simulink model "Main"  (R2025a)
settings: Solver=VariableStepAuto  StartTime=0.0  StopTime=inf  RelTol=1e-3
libraries: dspstat3 x21, simulink_extras x2, fuzblock x1
settings Model: Creator=felix  LastModifiedBy=felix

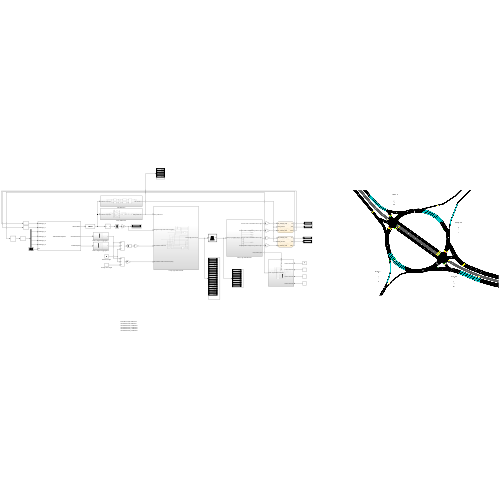
[thumbnail: Simulink's stored preview of the top-level diagram]
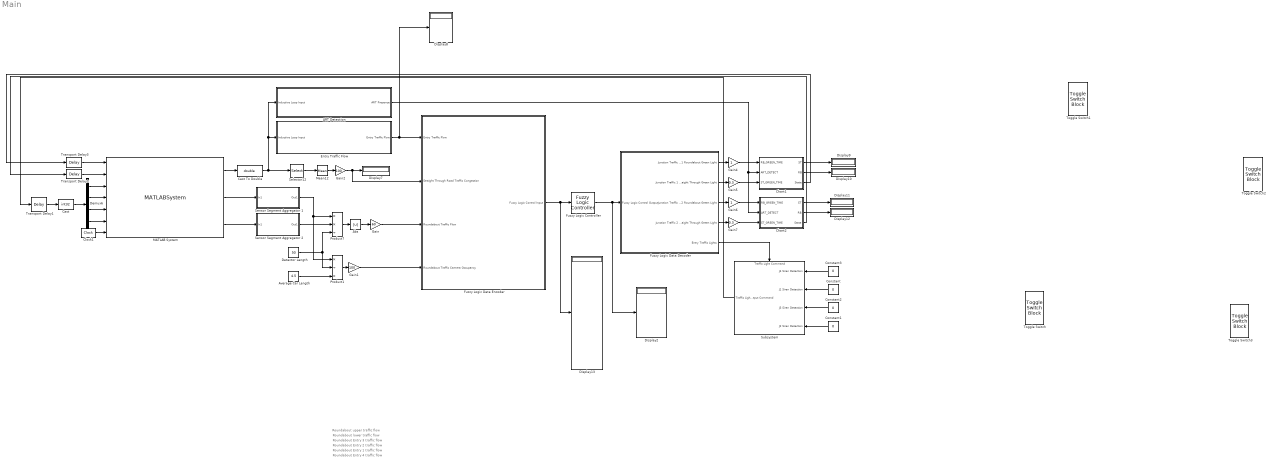
== system Main ==
  note: Roundabout Entry 4 traffic flow
  note: Roundabout Entry 1 traffic flow
  note: Roundabout Entry 2 traffic flow
  note: Roundabout Entry 3 traffic flow
  note: Roundabout lower traffic flow
  note: Roundabout upper traffic flow
  ART Detection : Subsystem
  Abs : Abs  SaturateOnIntegerOverflow=off
  Average Car Length : Constant  Value=4.5
  Cast : DataTypeConversion  OutDataTypeStr=int32  SaturateOnIntegerOverflow=off  RndMeth=Floor
  Cast To Double : DataTypeConversion  OutDataTypeStr=double  SaturateOnIntegerOverflow=off  RndMeth=Floor
  Chart1 : Stateflow chart  TreatAsAtomicUnit=on
      settings: PortSchema="{\"entries\":[{\"content\":{\"sides\":[{\"content\":{\"connectorIds\":[\"In1\",\"In3\",\"In2\"]},\"type\":\"ConnectorPlacement.EquallySpacedRectSide\",\"uuid\":\"637e66cb-ca59-4601-bc87-d398030e3d4e\"},{\"content\":{\"connectorIds\":[\"Out1\",\"Out2\",\"Out3\"],\"side\":\"RIGHT\"},\"type\":\"ConnectorPlacement.EquallySpacedRectSide\",\"uuid\":\"e38eed65-4b8e-4656-a325-0944c1a393f4\"},{\"content\":{\"side\":\"TOP\"},\"type\":\"ConnectorPlacement.EquallySpacedRectSide\",\"uuid\":\"0e3a8e04-edc4-4c67-baf8-ce5088455846\"}]},\"type\":\"ConnectorPlacement.EquallySpacedConnector\",\"uuid\":\"3222c7f8-a245-402d-95e3-93e9ec8df21d\"}],\"packageUris\":[\"http://schema.mathworks.com/mf0/Connector/R2020b\"],\"version\":\"1.0\"}"
  Chart2 : Stateflow chart  TreatAsAtomicUnit=on
      settings: PortSchema="{\"entries\":[{\"content\":{\"sides\":[{\"content\":{\"connectorIds\":[\"In1\",\"In3\",\"In2\"]},\"type\":\"ConnectorPlacement.EquallySpacedRectSide\",\"uuid\":\"3ce13be8-2b6b-44a6-8be1-1e74bcb078bf\"},{\"content\":{\"connectorIds\":[\"Out1\",\"Out2\",\"Out3\"],\"side\":\"RIGHT\"},\"type\":\"ConnectorPlacement.EquallySpacedRectSide\",\"uuid\":\"50de3ca6-7955-42e3-b87c-50e859948895\"},{\"content\":{\"side\":\"TOP\"},\"type\":\"ConnectorPlacement.EquallySpacedRectSide\",\"uuid\":\"25d95324-83a1-4a5c-ac4a-89a957fffa35\"}]},\"type\":\"ConnectorPlacement.EquallySpacedConnector\",\"uuid\":\"16ab9be5-7112-4953-b8f3-ef270fba1945\"}],\"packageUris\":[\"http://schema.mathworks.com/mf0/Connector/R2020b\"],\"version\":\"1.0\"}"
  Clock1 : simulink_extras/Flip Flops/Clock  period=1
  Constant{,1..3} (4 alike) : Constant  Value=0
  Demux6 : Demux
  Detector Length : Constant  Value=50
  Display{2,7..13} (8 alike) : Display
  Entry Traffic Flow : Subsystem
  Fuzzy Logic Controller : fuzblock/Fuzzy Logic  Controller  FIS='ComplexIntersectionFLC.fis'  OutputSampleNumber=101  DataType=double  UseLookupTable=off  NumBreakpoints=10  FuzzifiedInputs=off  RuleFiringStrengths=off  RuleOutputs=off  AggregatedOutputs=off  SimulateUsing=Code generation  OutOfRangeInputValueMessage=warning  NoRuleFiredMessage=warning  EmptyOutputFuzzySetMessage=warning
  Fuzzy Logic Data Decoder : Subsystem
  Fuzzy Logic Data Encoder : Subsystem
  Gain : Gain  Gain=60
  Gain1 : Gain  Gain=100
  Gain2 : Gain  Gain=100
  Gain4 : Gain
  Gain5 : Gain  Gain=0.3
  Gain6 : Gain
  Gain7 : Gain  Gain=0.3
  MATLAB System : MATLABSystem  System=TrafficSimulationSystem  Host=127.0.0.1  Port=55000  NumDetectors=29  NumAreaDetectors=13  NumTrafficLights=6  SimulateUsing=Interpreted execution
      mask Type: TrafficSimulationSystem
  Mean12 : dspstat3/Mean  run=off  InputProcessing=Columns as channels (frame based)  reset_popup=None  directionMode=Each column  dimension=1  roiEnable=off  roiType=Rectangles  roiPortion=Entire ROI  roiOutput=Individual statistics for each ROI  roiFlag=off  roundingMode=Floor  overflowMode=off  outputDataTypeStr=Inherit: Same as accumulator  outputMin=[]  outputMax=[]  outputLastDataTypeStr=Inherit: Same as accumulator
  Product1 : Product  Inputs=*/*
  Product7 : Product  Inputs=**/
  Selector12 : Selector  InputPortWidth=29  IndexOptions=Index vector (dialog)  Indices=[23 22 6 5]  OutputSizes=1
  Sensor Segment Aggregator 1 : Subsystem
  Sensor Segment Aggregator 2 : Subsystem
  Subsystem : Subsystem
      settings: PortSchema="{\"entries\":[{\"content\":{\"sides\":[{\"content\":{\"connectorIds\":[\"Out1\"]},\"type\":\"ConnectorPlacement.EquallySpacedRectSide\",\"uuid\":\"0ab4d31f-6d8d-40cf-8f31-cc7b1981b576\"},{\"content\":{\"connectorIds\":[\"In2\",\"In3\",\"In4\",\"In5\"],\"side\":\"RIGHT\"},\"type\":\"ConnectorPlacement.EquallySpacedRectSide\",\"uuid\":\"18efa56d-c6e6-40cd-9e32-fb69fe289a7f\"},{\"content\":{\"connectorIds\":[\"In1\"],\"side\":\"TOP\"},\"type\":\"ConnectorPlacement.EquallySpacedRectSide\",\"uuid\":\"5df0eb61-2f00-4eb6-96c4-d63daa7aa2fe\"}]},\"type\":\"ConnectorPlacement.EquallySpacedConnector\",\"uuid\":\"16d61d6a-1108-4e13-b7a6-dfccb8557755\"}],\"packageUris\":[\"http://schema.mathworks.com/mf0/Connector/R2020b\"],\"version\":\"1.0\"}"
  Toggle Switch{,1..3} (4 alike) : ToggleSwitchBlock
  Transport Delay1 : TransportDelay
  Transport Delay2 : TransportDelay
  Transport Delay3 : TransportDelay
  wires:
  MATLAB System/1 -> Cast To Double/1
  Product7/1 -> Abs/1
  Abs/1 -> Gain/1
  Fuzzy Logic Controller/1 -> Display2/1, Fuzzy Logic Data Decoder/1(Fuzzy Logic Control Output)
  Detector Length/1 -> Product7/3, Product1/2
  Average Car Length/1 -> Product1/3
  Product1/1 -> Gain1/1
  Selector12/1 -> Mean12/1
  Cast To Double/1 -> Selector12/1, ART Detection/1(Inductive Loop Input), Entry Traffic Flow/1(Inductive Loop Input)
  Mean12/1 -> Gain2/1
  Gain2/1 -> Display7/1, Fuzzy Logic Data Encoder/2(Straight Through Road Traffic Congestion)
  Gain5/1 -> Chart1/2(ST_GREEN_TIME)
  Gain4/1 -> Chart1/1(RB_GREEN_TIME)
  Gain6/1 -> Chart2/1(RB_GREEN_TIME)
  Gain7/1 -> Chart2/2(ST_GREEN_TIME)
  Clock1/1 -> MATLAB System/7
  Transport Delay3/1 -> MATLAB System/1
  Transport Delay2/1 -> MATLAB System/2
  Demux6/1 -> MATLAB System/3
  Demux6/2 -> MATLAB System/4
  Demux6/3 -> MATLAB System/5
  Demux6/4 -> MATLAB System/6
  Transport Delay1/1 -> Cast/1
  Cast/1 -> Demux6/1
  Chart1/3(State) -> Transport Delay3/1
  Chart2/3(State) -> Transport Delay2/1
  Chart1/1(ST) -> Display9/1
  Chart1/2(RB) -> Display10/1
  Chart2/1(ST) -> Display11/1
  Chart2/2(RB) -> Display12/1
  Sensor Segment Aggregator 1/1(Out1) -> Product7/1, Product1/1
  MATLAB System/2 -> Sensor Segment Aggregator 1/1(In1)
  Sensor Segment Aggregator 2/1(Out1) -> Product7/2
  MATLAB System/3 -> Sensor Segment Aggregator 2/1(In1)
  Fuzzy Logic Data Encoder/1(Fuzzy Logic Control Input) -> Display13/1, Fuzzy Logic Controller/1
  Gain/1 -> Fuzzy Logic Data Encoder/3(Roundabout Traffic Flow)
  Fuzzy Logic Data Decoder/1(Junction Traffic 1 Roundabout Green Light) -> Gain4/1
  Fuzzy Logic Data Decoder/2(Junction Traffic 1 Straight Through Green Light) -> Gain5/1
  Fuzzy Logic Data Decoder/3(Junction Traffic 2 Roundabout Green Light) -> Gain6/1
  Fuzzy Logic Data Decoder/4(Junction Traffic 2 Straight Through Green Light) -> Gain7/1
  Fuzzy Logic Data Decoder/5(Entry Traffic Lights) -> Subsystem/1(Traffic Light Command)
  Constant/1 -> Subsystem/3(J1 Siren Detection)
  Constant1/1 -> Subsystem/5(J2 Siren Detection)
  Constant2/1 -> Subsystem/4(J3 Siren Detection)
  Constant3/1 -> Subsystem/2(J4 Siren Detection)
  Subsystem/1(Traffic Light Output Command) -> Transport Delay1/1
  Gain1/1 -> Fuzzy Logic Data Encoder/4(Roundabout Traffic Camera Occupancy)
  ART Detection/1(ART Presence) -> Chart1/3(ART_DETECT), Chart2/3(ART_DETECT)
  Entry Traffic Flow/1(Entry Traffic Flow) -> Fuzzy Logic Data Encoder/1(Entry Traffic Flow), Display8/1

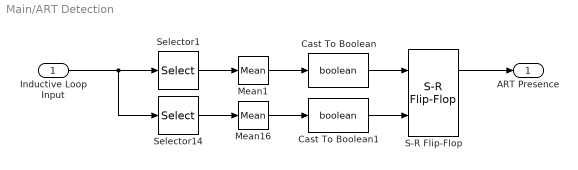
== system Main/ART Detection ==
  Inductive Loop Input : Inport
  Cast To Boolean : DataTypeConversion  OutDataTypeStr=boolean  SaturateOnIntegerOverflow=off  RndMeth=Floor
  Cast To Boolean1 : DataTypeConversion  OutDataTypeStr=boolean  SaturateOnIntegerOverflow=off  RndMeth=Floor
  Mean1 : dspstat3/Mean  run=off  InputProcessing=Columns as channels (frame based)  reset_popup=None  directionMode=Each column  dimension=1  roiEnable=off  roiType=Rectangles  roiPortion=Entire ROI  roiOutput=Individual statistics for each ROI  roiFlag=off  roundingMode=Floor  overflowMode=off  outputDataTypeStr=Inherit: Same as accumulator  outputMin=[]  outputMax=[]  outputLastDataTypeStr=Inherit: Same as accumulator
  Mean16 : dspstat3/Mean  run=off  InputProcessing=Columns as channels (frame based)  reset_popup=None  directionMode=Each column  dimension=1  roiEnable=off  roiType=Rectangles  roiPortion=Entire ROI  roiOutput=Individual statistics for each ROI  roiFlag=off  roundingMode=Floor  overflowMode=off  outputDataTypeStr=Inherit: Same as accumulator  outputMin=[]  outputMax=[]  outputLastDataTypeStr=Inherit: Same as accumulator
  S-R Flip-Flop : simulink_extras/Flip Flops/S-R Flip-Flop  initial_condition=0
  Selector1 : Selector  InputPortWidth=29  IndexOptions=Index vector (dialog)  Indices=[29 28]  OutputSizes=1
  Selector14 : Selector  InputPortWidth=29  IndexOptions=Index vector (dialog)  Indices=[21 20]  OutputSizes=1
  ART Presence : Outport
  wires:
  Mean16/1 -> Cast To Boolean1/1
  Cast To Boolean1/1 -> S-R Flip-Flop/2
  Selector1/1 -> Mean1/1
  Inductive Loop Input/1 -> Selector14/1, Selector1/1
  Mean1/1 -> Cast To Boolean/1
  Selector14/1 -> Mean16/1
  Cast To Boolean/1 -> S-R Flip-Flop/1
  S-R Flip-Flop/1 -> ART Presence/1

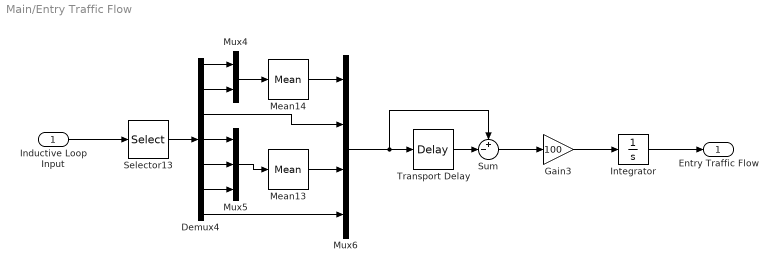
== system Main/Entry Traffic Flow ==
  Inductive Loop Input : Inport
  Demux4 : Demux  Outputs=7
  Gain3 : Gain  Gain=100
  Integrator : Integrator
  Mean13 : dspstat3/Mean  run=off  InputProcessing=Columns as channels (frame based)  reset_popup=None  directionMode=Each column  dimension=1  roiEnable=off  roiType=Rectangles  roiPortion=Entire ROI  roiOutput=Individual statistics for each ROI  roiFlag=off  roundingMode=Floor  overflowMode=off  outputDataTypeStr=Inherit: Same as accumulator  outputMin=[]  outputMax=[]  outputLastDataTypeStr=Inherit: Same as accumulator
  Mean14 : dspstat3/Mean  run=off  InputProcessing=Columns as channels (frame based)  reset_popup=None  directionMode=Each column  dimension=1  roiEnable=off  roiType=Rectangles  roiPortion=Entire ROI  roiOutput=Individual statistics for each ROI  roiFlag=off  roundingMode=Floor  overflowMode=off  outputDataTypeStr=Inherit: Same as accumulator  outputMin=[]  outputMax=[]  outputLastDataTypeStr=Inherit: Same as accumulator
  Mux4 : Mux  Inputs=2
  Mux5 : Mux  Inputs=3
  Mux6 : Mux
  Selector13 : Selector  InputPortWidth=29  IndexOptions=Index vector (dialog)  Indices=[10 11 17 14 15 16 12]  OutputSizes=1
  Sum : Sum  Inputs=+-|
  Transport Delay : TransportDelay  DelayTime=10  BufferSize=4000
  Entry Traffic Flow : Outport
  wires:
  Demux4/2 -> Mux4/2
  Demux4/5 -> Mux5/2
  Demux4/4 -> Mux5/1
  Selector13/1 -> Demux4/1
  Mean13/1 -> Mux6/3
  Sum/1 -> Gain3/1
  Demux4/3 -> Mux6/2
  Mux6/1 -> Sum/1, Transport Delay/1
  Demux4/1 -> Mux4/1
  Mean14/1 -> Mux6/1
  Transport Delay/1 -> Sum/2
  Demux4/7 -> Mux6/4
  Mux5/1 -> Mean13/1
  Demux4/6 -> Mux5/3
  Mux4/1 -> Mean14/1
  Gain3/1 -> Integrator/1
  Integrator/1 -> Entry Traffic Flow/1
  Inductive Loop Input/1 -> Selector13/1

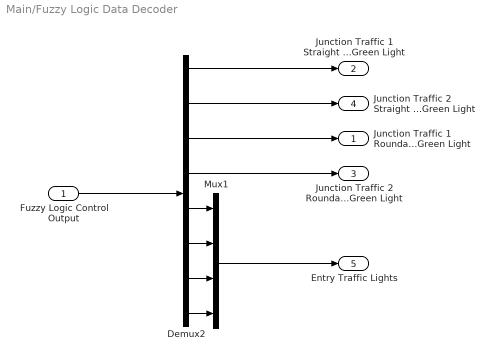
== system Main/Fuzzy Logic Data Decoder ==
  Fuzzy Logic Control Output : Inport
  Demux2 : Demux  Outputs=8
  Mux1 : Mux
  Junction Traffic 1 Roundabout Green Light : Outport
  Junction Traffic 1 Straight Through Green Light : Outport  Port=2
  Junction Traffic 2 Roundabout Green Light : Outport  Port=3
  Junction Traffic 2 Straight Through Green Light : Outport  Port=4
  Entry Traffic Lights : Outport  Port=5
  wires:
  Demux2/6 -> Mux1/2
  Fuzzy Logic Control Output/1 -> Demux2/1
  Demux2/4 -> Junction Traffic 2 Roundabout Green Light/1
  Demux2/7 -> Mux1/3
  Demux2/5 -> Mux1/1
  Demux2/1 -> Junction Traffic 1 Straight Through Green Light/1
  Demux2/8 -> Mux1/4
  Mux1/1 -> Entry Traffic Lights/1
  Demux2/2 -> Junction Traffic 2 Straight Through Green Light/1
  Demux2/3 -> Junction Traffic 1 Roundabout Green Light/1

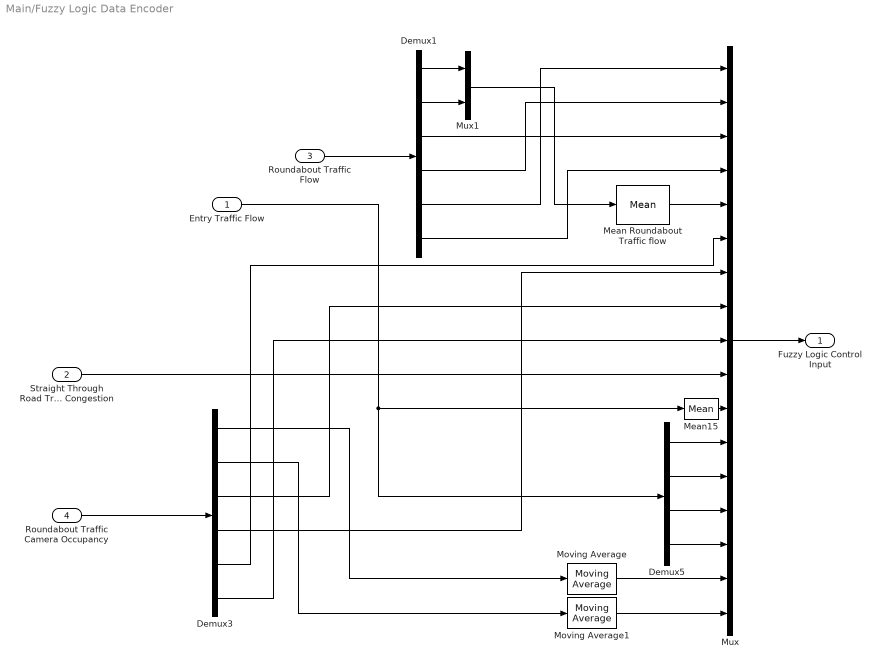
== system Main/Fuzzy Logic Data Encoder ==
  Entry Traffic Flow : Inport
  Straight Through Road Traffic Congestion : Inport  Port=2
  Roundabout Traffic Flow : Inport  Port=3
  Roundabout Traffic Camera Occupancy : Inport  Port=4
  Demux1 : Demux  Outputs=6
  Demux3 : Demux  Outputs=6
  Demux5 : Demux
  Mean Roundabout Traffic flow : dspstat3/Mean  run=off  InputProcessing=Columns as channels (frame based)  reset_popup=None  directionMode=Each column  dimension=1  roiEnable=off  roiType=Rectangles  roiPortion=Entire ROI  roiOutput=Individual statistics for each ROI  roiFlag=off  roundingMode=Floor  overflowMode=off  outputDataTypeStr=Inherit: Same as accumulator  outputMin=[]  outputMax=[]  outputLastDataTypeStr=Inherit: Same as accumulator
  Mean15 : dspstat3/Mean  run=off  InputProcessing=Columns as channels (frame based)  reset_popup=None  directionMode=Each column  dimension=1  roiEnable=off  roiType=Rectangles  roiPortion=Entire ROI  roiOutput=Individual statistics for each ROI  roiFlag=off  roundingMode=Floor  overflowMode=off  outputDataTypeStr=Inherit: Same as accumulator  outputMin=[]  outputMax=[]  outputLastDataTypeStr=Inherit: Same as accumulator
  Moving Average : dspstat3/Moving Average  Method=Exponential weighting  ForgettingFactorPort=off  SpecifyWindowLength=off  WindowLength=12  OverlapLength=3  AllowArbitraryInputLength=off  ForgettingFactor=0.9  SimulateUsing=Code generation
  Moving Average1 : dspstat3/Moving Average  Method=Exponential weighting  ForgettingFactorPort=off  SpecifyWindowLength=off  WindowLength=12  OverlapLength=3  AllowArbitraryInputLength=off  ForgettingFactor=0.9  SimulateUsing=Code generation
  Mux : Mux  Inputs=17
  Mux1 : Mux  Inputs=2
  Fuzzy Logic Control Input : Outport
  wires:
  Demux1/3 -> Mux/3
  Demux1/2 -> Mux1/2
  Demux3/3 -> Mux/8
  Demux3/4 -> Mux/7
  Demux3/6 -> Mux/9
  Demux5/4 -> Mux/15
  Demux3/5 -> Mux/6
  Straight Through Road Traffic Congestion/1 -> Mux/10
  Moving Average/1 -> Mux/16
  Mux1/1 -> Mean Roundabout Traffic flow/1
  Demux5/2 -> Mux/13
  Demux3/1 -> Moving Average/1
  Mean Roundabout Traffic flow/1 -> Mux/5
  Roundabout Traffic Camera Occupancy/1 -> Demux3/1
  Mean15/1 -> Mux/11
  Demux3/2 -> Moving Average1/1
  Demux1/5 -> Mux/1
  Demux1/4 -> Mux/2
  Demux5/1 -> Mux/12
  Demux1/1 -> Mux1/1
  Entry Traffic Flow/1 -> Demux5/1, Mean15/1
  Demux1/6 -> Mux/4
  Demux5/3 -> Mux/14
  Moving Average1/1 -> Mux/17
  Mux/1 -> Fuzzy Logic Control Input/1
  Roundabout Traffic Flow/1 -> Demux1/1

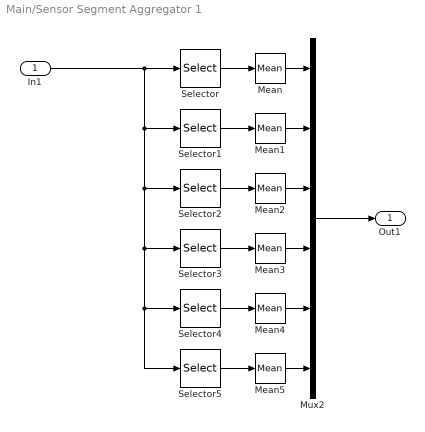
== system Main/Sensor Segment Aggregator 1 ==
  In1 : Inport
  Mean{,1..5} (6 alike) : dspstat3/Mean  run=off  InputProcessing=Columns as channels (frame based)  reset_popup=None  directionMode=Each column  dimension=1  roiEnable=off  roiType=Rectangles  roiPortion=Entire ROI  roiOutput=Individual statistics for each ROI  roiFlag=off  roundingMode=Floor  overflowMode=off  outputDataTypeStr=Inherit: Same as accumulator  outputMin=[]  outputMax=[]  outputLastDataTypeStr=Inherit: Same as accumulator
  Mux2 : Mux  Inputs=6
  Selector : Selector  InputPortWidth=13  IndexOptions=Index vector (dialog)  Indices=[1 2 6]  OutputSizes=1
  Selector1 : Selector  InputPortWidth=13  IndexOptions=Index vector (dialog)  Indices=[7 8 9]  OutputSizes=1
  Selector2 : Selector  InputPortWidth=13  IndexOptions=Index vector (dialog)  Indices=[10 11 12]  OutputSizes=1
  Selector3 : Selector  InputPortWidth=13  IndexOptions=Index vector (dialog)  Indices=[13]  OutputSizes=1
  Selector4 : Selector  InputPortWidth=13  IndexOptions=Index vector (dialog)  Indices=[3 4]  OutputSizes=1
  Selector5 : Selector  InputPortWidth=13  IndexOptions=Index vector (dialog)  Indices=[5]  OutputSizes=1
  Out1 : Outport
  wires:
  Mean5/1 -> Mux2/6
  Mean3/1 -> Mux2/4
  Mux2/1 -> Out1/1
  Selector4/1 -> Mean4/1
  Mean2/1 -> Mux2/3
  In1/1 -> Selector5/1, Selector4/1, Selector3/1, Selector2/1, Selector1/1, Selector/1
  Selector/1 -> Mean/1
  Selector1/1 -> Mean1/1
  Selector3/1 -> Mean3/1
  Selector2/1 -> Mean2/1
  Mean4/1 -> Mux2/5
  Mean/1 -> Mux2/1
  Selector5/1 -> Mean5/1
  Mean1/1 -> Mux2/2

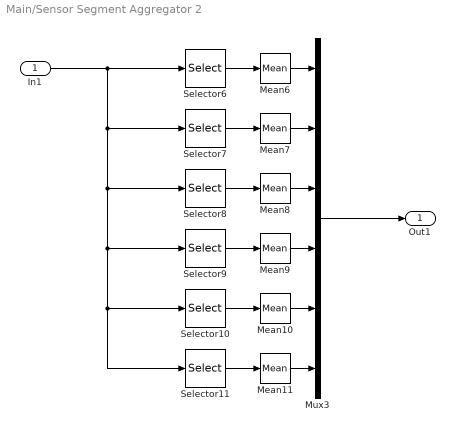
== system Main/Sensor Segment Aggregator 2 ==
  In1 : Inport
  Mean{6..11} (6 alike) : dspstat3/Mean  run=off  InputProcessing=Columns as channels (frame based)  reset_popup=None  directionMode=Each column  dimension=1  roiEnable=off  roiType=Rectangles  roiPortion=Entire ROI  roiOutput=Individual statistics for each ROI  roiFlag=off  roundingMode=Floor  overflowMode=off  outputDataTypeStr=Inherit: Same as accumulator  outputMin=[]  outputMax=[]  outputLastDataTypeStr=Inherit: Same as accumulator
  Mux3 : Mux  Inputs=6
  Selector10 : Selector  InputPortWidth=13  IndexOptions=Index vector (dialog)  Indices=[3 4]  OutputSizes=1
  Selector11 : Selector  InputPortWidth=13  IndexOptions=Index vector (dialog)  Indices=[5]  OutputSizes=1
  Selector6 : Selector  InputPortWidth=13  IndexOptions=Index vector (dialog)  Indices=[1 2 6]  OutputSizes=1
  Selector7 : Selector  InputPortWidth=13  IndexOptions=Index vector (dialog)  Indices=[7 8 9]  OutputSizes=1
  Selector8 : Selector  InputPortWidth=13  IndexOptions=Index vector (dialog)  Indices=[10 11 12]  OutputSizes=1
  Selector9 : Selector  InputPortWidth=13  IndexOptions=Index vector (dialog)  Indices=[13]  OutputSizes=1
  Out1 : Outport
  wires:
  In1/1 -> Selector6/1, Selector7/1, Selector8/1, Selector9/1, Selector10/1, Selector11/1
  Selector11/1 -> Mean11/1
  Selector6/1 -> Mean6/1
  Selector8/1 -> Mean8/1
  Mean11/1 -> Mux3/6
  Selector10/1 -> Mean10/1
  Mean10/1 -> Mux3/5
  Selector9/1 -> Mean9/1
  Mean9/1 -> Mux3/4
  Mean8/1 -> Mux3/3
  Mean6/1 -> Mux3/1
  Selector7/1 -> Mean7/1
  Mean7/1 -> Mux3/2
  Mux3/1 -> Out1/1

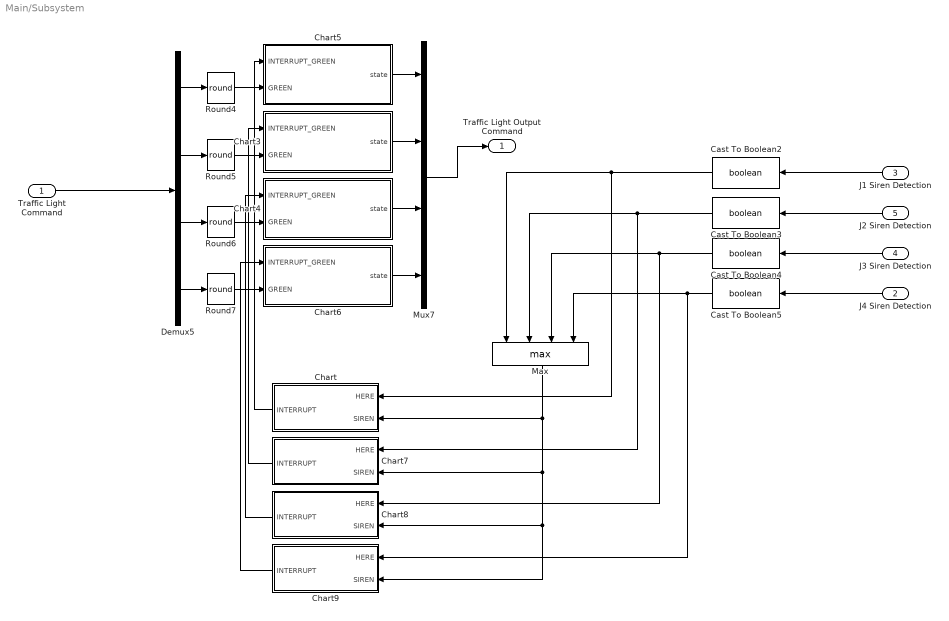
== system Main/Subsystem ==
  Traffic Light Command : Inport
  J4 Siren Detection : Inport  Port=2
  J1 Siren Detection : Inport  Port=3
  J3 Siren Detection : Inport  Port=4
  J2 Siren Detection : Inport  Port=5
  Cast To Boolean{2..5} (4 alike) : DataTypeConversion  OutDataTypeStr=boolean  SaturateOnIntegerOverflow=off  RndMeth=Floor
  Chart : Stateflow chart  TreatAsAtomicUnit=on
  Chart3 : Stateflow chart  TreatAsAtomicUnit=on
      settings: PortSchema="{\"entries\":[{\"content\":{\"sides\":[{\"content\":{\"connectorIds\":[\"In2\",\"In1\"]},\"type\":\"ConnectorPlacement.EquallySpacedRectSide\",\"uuid\":\"47c49a95-aba9-457a-82de-dbe7ab38dc2f\"},{\"content\":{\"connectorIds\":[\"Out1\"],\"side\":\"RIGHT\"},\"type\":\"ConnectorPlacement.EquallySpacedRectSide\",\"uuid\":\"31393c1e-4f20-4a35-8dbf-34cba7a73095\"},{\"content\":{\"side\":\"TOP\"},\"type\":\"ConnectorPlacement.EquallySpacedRectSide\",\"uuid\":\"f18f7e9b-4e01-4aa3-9e9a-2ba33b411dff\"}]},\"type\":\"ConnectorPlacement.EquallySpacedConnector\",\"uuid\":\"856e1e73-fa54-45f8-9e7d-91d6401f4c99\"}],\"packageUris\":[\"http://schema.mathworks.com/mf0/Connector/R2020b\"],\"version\":\"1.0\"}"
  Chart4 : Stateflow chart  TreatAsAtomicUnit=on
      settings: PortSchema="{\"entries\":[{\"content\":{\"sides\":[{\"content\":{\"connectorIds\":[\"In2\",\"In1\"]},\"type\":\"ConnectorPlacement.EquallySpacedRectSide\",\"uuid\":\"47c49a95-aba9-457a-82de-dbe7ab38dc2f\"},{\"content\":{\"connectorIds\":[\"Out1\"],\"side\":\"RIGHT\"},\"type\":\"ConnectorPlacement.EquallySpacedRectSide\",\"uuid\":\"31393c1e-4f20-4a35-8dbf-34cba7a73095\"},{\"content\":{\"side\":\"TOP\"},\"type\":\"ConnectorPlacement.EquallySpacedRectSide\",\"uuid\":\"f18f7e9b-4e01-4aa3-9e9a-2ba33b411dff\"}]},\"type\":\"ConnectorPlacement.EquallySpacedConnector\",\"uuid\":\"856e1e73-fa54-45f8-9e7d-91d6401f4c99\"}],\"packageUris\":[\"http://schema.mathworks.com/mf0/Connector/R2020b\"],\"version\":\"1.0\"}"
  Chart5 : Stateflow chart  TreatAsAtomicUnit=on
      settings: PortSchema="{\"entries\":[{\"content\":{\"sides\":[{\"content\":{\"connectorIds\":[\"In2\",\"In1\"]},\"type\":\"ConnectorPlacement.EquallySpacedRectSide\",\"uuid\":\"47c49a95-aba9-457a-82de-dbe7ab38dc2f\"},{\"content\":{\"connectorIds\":[\"Out1\"],\"side\":\"RIGHT\"},\"type\":\"ConnectorPlacement.EquallySpacedRectSide\",\"uuid\":\"31393c1e-4f20-4a35-8dbf-34cba7a73095\"},{\"content\":{\"side\":\"TOP\"},\"type\":\"ConnectorPlacement.EquallySpacedRectSide\",\"uuid\":\"f18f7e9b-4e01-4aa3-9e9a-2ba33b411dff\"}]},\"type\":\"ConnectorPlacement.EquallySpacedConnector\",\"uuid\":\"856e1e73-fa54-45f8-9e7d-91d6401f4c99\"}],\"packageUris\":[\"http://schema.mathworks.com/mf0/Connector/R2020b\"],\"version\":\"1.0\"}"
  Chart6 : Stateflow chart  TreatAsAtomicUnit=on
      settings: PortSchema="{\"entries\":[{\"content\":{\"sides\":[{\"content\":{\"connectorIds\":[\"In2\",\"In1\"]},\"type\":\"ConnectorPlacement.EquallySpacedRectSide\",\"uuid\":\"47c49a95-aba9-457a-82de-dbe7ab38dc2f\"},{\"content\":{\"connectorIds\":[\"Out1\"],\"side\":\"RIGHT\"},\"type\":\"ConnectorPlacement.EquallySpacedRectSide\",\"uuid\":\"31393c1e-4f20-4a35-8dbf-34cba7a73095\"},{\"content\":{\"side\":\"TOP\"},\"type\":\"ConnectorPlacement.EquallySpacedRectSide\",\"uuid\":\"f18f7e9b-4e01-4aa3-9e9a-2ba33b411dff\"}]},\"type\":\"ConnectorPlacement.EquallySpacedConnector\",\"uuid\":\"856e1e73-fa54-45f8-9e7d-91d6401f4c99\"}],\"packageUris\":[\"http://schema.mathworks.com/mf0/Connector/R2020b\"],\"version\":\"1.0\"}"
  Chart7 : Stateflow chart  TreatAsAtomicUnit=on
  Chart8 : Stateflow chart  TreatAsAtomicUnit=on
  Chart9 : Stateflow chart  TreatAsAtomicUnit=on
  Demux5 : Demux
  Max : MinMax  Function=max  Inputs=4
  Mux7 : Mux
  Round{4..7} (4 alike) : Rounding  Operator=round
  Traffic Light Output Command : Outport
  wires:
  Chart7/1(INTERRUPT) -> Chart3/2(INTERRUPT_GREEN)
  Chart8/1(INTERRUPT) -> Chart4/2(INTERRUPT_GREEN)
  Cast To Boolean3/1 -> Chart7/1(HERE), Max/2
  Max/1 -> Chart9/2(SIREN), Chart8/2(SIREN), Chart7/2(SIREN), Chart/2(SIREN)
  Demux5/4 -> Round7/1
  J1 Siren Detection/1 -> Cast To Boolean2/1
  J3 Siren Detection/1 -> Cast To Boolean4/1
  Cast To Boolean2/1 -> Chart/1(HERE), Max/1
  Round6/1 -> Chart4/1(GREEN)
  Cast To Boolean5/1 -> Chart9/1(HERE), Max/4
  Cast To Boolean4/1 -> Max/3, Chart8/1(HERE)
  Demux5/1 -> Round4/1
  J4 Siren Detection/1 -> Cast To Boolean5/1
  Chart4/1(state) -> Mux7/3
  Chart9/1(INTERRUPT) -> Chart6/2(INTERRUPT_GREEN)
  Round7/1 -> Chart6/1(GREEN)
  Demux5/2 -> Round5/1
  Chart5/1(state) -> Mux7/1
  Chart3/1(state) -> Mux7/2
  Chart6/1(state) -> Mux7/4
  Chart/1(INTERRUPT) -> Chart5/2(INTERRUPT_GREEN)
  Round4/1 -> Chart5/1(GREEN)
  Demux5/3 -> Round6/1
  Round5/1 -> Chart3/1(GREEN)
  Mux7/1 -> Traffic Light Output Command/1
  J2 Siren Detection/1 -> Cast To Boolean3/1
  Traffic Light Command/1 -> Demux5/1

== stateflow chart Main/Subsystem/Chart4 ==
  settings: stateMachineType=MOORE_MACHINE  executeAtInitialization=1
  state Yellow1
    state=1;
  state Green
    state=0;
  state Red
    state=2;
  state Yellow2
    state=1;
  Green -> Yellow1 : [GREEN==0||INTERRUPT_GREEN==2]
  Yellow1 -> Red : [after(1, sec)]
  (default) -> Green
  Red -> Green [order 2] : [INTERRUPT_GREEN==1]
  Yellow2 -> Green : [after(1, sec)]
  Red -> Yellow2 [order 1] : [GREEN==1&&INTERRUPT_GREEN!=2]
  data: state output double; GREEN input; INTERRUPT_GREEN input

== stateflow chart Main/Subsystem/Chart6 ==
  settings: stateMachineType=MOORE_MACHINE  executeAtInitialization=1
  state Yellow1
    state=1;
  state Green
    state=0;
  state Red
    state=2;
  state Yellow2
    state=1;
  Green -> Yellow1 : [GREEN==0||INTERRUPT_GREEN==2]
  Yellow1 -> Red : [after(1, sec)]
  (default) -> Green
  Red -> Green [order 2] : [INTERRUPT_GREEN==1]
  Yellow2 -> Green : [after(1, sec)]
  Red -> Yellow2 [order 1] : [GREEN==1&&INTERRUPT_GREEN!=2]
  data: state output double; GREEN input; INTERRUPT_GREEN input

== stateflow chart Main/Subsystem/Chart5 ==
  settings: stateMachineType=MOORE_MACHINE  executeAtInitialization=1
  state Yellow1
    state=1;
  state Green
    state=0;
  state Red
    state=2;
  state Yellow2
    state=1;
  Green -> Yellow1 : [GREEN==0||INTERRUPT_GREEN==2]
  Yellow1 -> Red : [after(1, sec)]
  (default) -> Green
  Red -> Green [order 2] : [INTERRUPT_GREEN==1]
  Yellow2 -> Green : [after(1, sec)]
  Red -> Yellow2 [order 1] : [GREEN==1&&INTERRUPT_GREEN!=2]
  data: state output double; GREEN input; INTERRUPT_GREEN input

== stateflow chart Main/Subsystem/Chart ==
  settings: stateMachineType=MOORE_MACHINE  executeAtInitialization=1
  state INTERRUPT_RED
    INTERRUPT=2;
  state NORMAL
    INTERRUPT=0;
  state INTERRUPT_GREEN
    INTERRUPT=1;
  (default) -> NORMAL
  INTERRUPT_RED -> NORMAL : [SIREN==0]
  INTERRUPT_GREEN -> NORMAL : [SIREN==0]
  NORMAL -> INTERRUPT_GREEN [order 1] : [SIREN==1&&HERE==1]
  NORMAL -> INTERRUPT_RED [order 2] : [SIREN==1&&HERE==0]
  data: INTERRUPT output double; HERE input; SIREN input

== stateflow chart Main/Subsystem/Chart7 ==
  settings: stateMachineType=MOORE_MACHINE  executeAtInitialization=1
  state INTERRUPT_RED
    INTERRUPT=2;
  state NORMAL
    INTERRUPT=0;
  state INTERRUPT_GREEN
    INTERRUPT=1;
  (default) -> NORMAL
  INTERRUPT_RED -> NORMAL : [SIREN==0]
  INTERRUPT_GREEN -> NORMAL : [SIREN==0]
  NORMAL -> INTERRUPT_GREEN [order 1] : [SIREN==1&&HERE==1]
  NORMAL -> INTERRUPT_RED [order 2] : [SIREN==1&&HERE==0]
  data: INTERRUPT output double; HERE input; SIREN input

== stateflow chart Main/Subsystem/Chart8 ==
  settings: stateMachineType=MOORE_MACHINE  executeAtInitialization=1
  state INTERRUPT_RED
    INTERRUPT=2;
  state NORMAL
    INTERRUPT=0;
  state INTERRUPT_GREEN
    INTERRUPT=1;
  (default) -> NORMAL
  INTERRUPT_RED -> NORMAL : [SIREN==0]
  INTERRUPT_GREEN -> NORMAL : [SIREN==0]
  NORMAL -> INTERRUPT_GREEN [order 1] : [SIREN==1&&HERE==1]
  NORMAL -> INTERRUPT_RED [order 2] : [SIREN==1&&HERE==0]
  data: INTERRUPT output double; HERE input; SIREN input

== stateflow chart Main/Subsystem/Chart9 ==
  settings: stateMachineType=MOORE_MACHINE  executeAtInitialization=1
  state INTERRUPT_RED
    INTERRUPT=2;
  state NORMAL
    INTERRUPT=0;
  state INTERRUPT_GREEN
    INTERRUPT=1;
  (default) -> NORMAL
  INTERRUPT_RED -> NORMAL : [SIREN==0]
  INTERRUPT_GREEN -> NORMAL : [SIREN==0]
  NORMAL -> INTERRUPT_GREEN [order 1] : [SIREN==1&&HERE==1]
  NORMAL -> INTERRUPT_RED [order 2] : [SIREN==1&&HERE==0]
  data: INTERRUPT output double; HERE input; SIREN input

== stateflow chart Main/Chart1 ==
  state RB_GREEN
    entry:
    RB=2;
    ST=0;
    State=3;
  state RB_YELLOW
    entry:
    RB=1;
    ST=0;
    State=4;
  state ALL_RED1
    entry:
    RB=0;
    ST=0;
    State=2;
  state ALL_RED
    entry:
    RB=0;
    ST=0;
    State=5;
  state ST_YELLOW
    entry:
    RB=0;
    ST=1;
    State=1;
  state ST_GREEN
    entry:
    RB=0;
    ST=2;
    State=0;
  (default) -> RB_GREEN
  RB_GREEN -> RB_YELLOW : [after(RB_GREEN_TIME, sec)||ART_DETECT>0.1]
  ALL_RED1 -> RB_GREEN [order 2] : [after(1, sec)]
  RB_YELLOW -> ALL_RED : [after(1, sec)]
  ALL_RED1 -> ST_GREEN [order 1] : [ART_DETECT>0.1]
  ST_YELLOW -> ALL_RED1 [order 2] : [after(2, sec)]
  ALL_RED -> ST_GREEN : [after(0.5, sec)]
  ST_GREEN -> ST_GREEN [order 1] : [ART_DETECT>0.1]
  ST_YELLOW -> ST_GREEN [order 1] : [ART_DETECT>0.1]
  ST_GREEN -> ST_YELLOW [order 3] : [after(ST_GREEN_TIME, sec)]
  ST_GREEN -> ST_YELLOW [order 2] : [ART_DETECT<0.1]
  data: ST output; RB output; RB_GREEN_TIME input; ST_GREEN_TIME input; State output double; ART_DETECT input

== stateflow chart Main/Chart2 ==
  state RB_GREEN
    entry:
    RB=2;
    ST=0;
    State=3;
  state RB_YELLOW
    entry:
    RB=1;
    ST=0;
    State=4;
  state ALL_RED1
    entry:
    RB=0;
    ST=0;
    State=2;
  state ALL_RED
    entry:
    RB=0;
    ST=0;
    State=5;
  state ST_YELLOW
    entry:
    RB=0;
    ST=1;
    State=1;
  state ST_GREEN
    entry:
    RB=0;
    ST=2;
    State=0;
  (default) -> RB_GREEN
  RB_GREEN -> RB_YELLOW : [after(RB_GREEN_TIME, sec)||ART_DETECT>0.1]
  ALL_RED1 -> RB_GREEN [order 2] : [after(1, sec)]
  RB_YELLOW -> ALL_RED : [after(1, sec)]
  ALL_RED1 -> ST_GREEN [order 1] : [ART_DETECT>0.1]
  ST_YELLOW -> ALL_RED1 [order 2] : [after(2, sec)]
  ALL_RED -> ST_GREEN : [after(0.5, sec)]
  ST_GREEN -> ST_GREEN [order 1] : [ART_DETECT>0.1]
  ST_YELLOW -> ST_GREEN [order 1] : [ART_DETECT>0.1]
  ST_GREEN -> ST_YELLOW [order 3] : [after(ST_GREEN_TIME, sec)]
  ST_GREEN -> ST_YELLOW [order 2] : [ART_DETECT<0.1]
  data: ST output; RB output; RB_GREEN_TIME input; ST_GREEN_TIME input; State output double; ART_DETECT input

== stateflow chart Main/Subsystem/Chart3 ==
  settings: stateMachineType=MOORE_MACHINE  executeAtInitialization=1
  state Yellow1
    state=1;
  state Green
    state=0;
  state Red
    state=2;
  state Yellow2
    state=1;
  Green -> Yellow1 : [GREEN==0||INTERRUPT_GREEN==2]
  Yellow1 -> Red : [after(1, sec)]
  (default) -> Green
  Red -> Green [order 2] : [INTERRUPT_GREEN==1]
  Yellow2 -> Green : [after(1, sec)]
  Red -> Yellow2 [order 1] : [GREEN==1&&INTERRUPT_GREEN!=2]
  data: state output double; GREEN input; INTERRUPT_GREEN input
